simulink model "serial_leg"  (R2025b)
settings: Solver=ode15s  StartTime=0.0  StopTime=50  MaxStep=1e-3  RelTol=1e-3
undefined symbols (not defined in the file): X, Y, Z
libraries: sm_lib x106, nesl_utility x25, slpidlib x2
(part 1 of 3)
settings Model: Creator=Hhop  LastModifiedBy=13302
settings SolverCC: AlgebraicLoopSolver=TrustRegion  MinimalZcImpactIntegration=on
settings DebuggingCC: ReadBeforeWriteMsg=DisableAll  WriteAfterWriteMsg=DisableAll  WriteAfterReadMsg=DisableAll  MultiTaskDSMMsg=none
settings ModelReferenceCC: UpdateModelReferenceTargets=IfOutOfDate
settings SFSimCC: SFSimEcho=off
settings RTWCC: GPUComputeCapability=3.5  DLArmComputeVersion=19.05

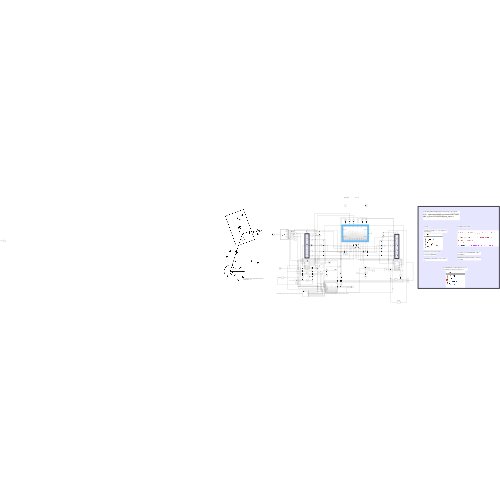
[thumbnail: Simulink's stored preview of the top-level diagram]
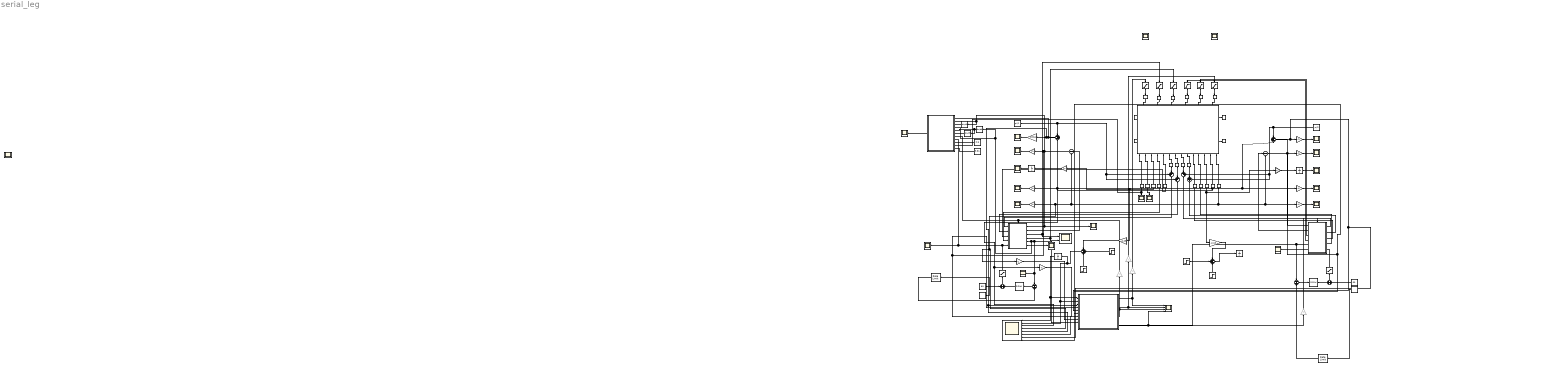
== system serial_leg ==
  note: 参考开源文档作者：韭菜的菜 链接：https://zhuanlan.zhihu.com/p/613007726 来源：知乎
  note: 图片来源 韭菜的菜 链接：https://zhuanlan.zhihu.com/p/613007726来源：知乎
  note: 运行步骤 :
  note: 所有开源文件必须置于同一文件夹(最好不要使用中文路径)
  note: 得到K参数后进入simulink 点击“运行”开始仿真
  note: addpath'(你所要想添加到的路径)'，具体用法可自行搜索
  note: 如果遇到如下图所示错误
  note: 可点击将其文件夹添加到MATLAB，或输入代码更换路径
  note: K = get_k_length(0.08)
  note: 在命令行窗口运行下图所示代码
  note: 如果想获取K矩阵关于腿长的函数的三次多项式系数在命令行窗口运行下图所示文件
  note: 该仿真是在b站轮腿机器人仿真开源上进行修改，链接：https://www.bilibili.com/read/cv26677904/?spm_id_from=333.999.0.0&jump_opus=1
  note: REAL serial/parallelogram mechanism: only A motors drive AD and AH. AD/AH use old upper-leg equivalent mass/inertia; DC/GHJ use old lower-leg equivalent mass/inertia. CEF and FG are transmission members with negligible mass. Original VMC and LQR are unchanged.
  Constant : Constant  Value=0.300
  Constant1 : Constant  Value=0.300
  Constant10 : Constant  Value=pi/2
  Constant12 : Constant  Value=pi/2
  Constant2 : Constant  Value=0.6
  Constant3 : Constant  Value=9.81
  Derivative : Derivative
  Derivative1 : Derivative
  Derivative2 : Derivative
  Gain : Gain  Gain=-0.08
  Gain1 : Gain  Gain=-0.05
  Gain{2..5} (4 alike) : Gain  Commented=through  Gain=-1
  Gain{22,24..26,33,36,38,40} (8 alike) : Gain  Gain=180/pi
  Gain29 : Gain  Gain=-0.0603
  Gain41 : Gain  Gain=-0.0603
  Gain6 : Gain  Gain=-1
  Gain7 : Gain  Gain=-1
  Integrator{1..4} (4 alike) : Integrator
  L_X : Scope
      settings: ActiveDisplayYMinimum=-0.7616  ActiveDisplayYMaximum=6.68295  DataLoggingVariableName=ScopeData7
  L_d_phi : Scope
      settings: ActiveDisplayYMinimum=-7.35816  ActiveDisplayYMaximum=0.81757  DataLoggingVariableName=ScopeData9
  L_d_theta : Scope
      settings: ActiveDisplayYMinimum=-21.72062  ActiveDisplayYMaximum=26.74747  DataLoggingVariableName=ScopeData13
  L_phi : Scope
      settings: ActiveDisplayYMinimum=-5.3646042462321226  ActiveDisplayYMaximum=10.928227501224146  DataLoggingVariableName=ScopeData22
  L_theta : Scope
      settings: ActiveDisplayYMinimum=-1.1015623623288358  ActiveDisplayYMaximum=1.79588161375989  DataLoggingVariableName=ScopeData25
  MATLAB Function : MATLAB Function  TreatAsAtomicUnit=on
  PID Controller2 : slpidlib/PID Controller  Controller=PID  Form=Parallel  TimeDomain=Continuous-time  UseExternalTs=off  SampleTime=-1  IntegratorMethod=Forward Euler  FilterMethod=Forward Euler  ControllerParametersSource=internal  P=500  I=0  UseKiTs=off  D=200  UseExternalDerivativeSource=off  N=100  UseFilter=on  TunerSelectOption=Transfer Function Based (PID Tuner App)  InitialConditionSource=internal  InitialConditionForIntegrator=0  InitialConditionForFilter=0  DifferentiatorICPrevScaledInput=0  ExternalReset=none  TrackingMode=off  Kt=1  LimitOutput=off  SatLimitsSource=internal  UpperSaturationLimit=inf  LowerSaturationLimit=-inf  LinearizeAsGain=on  AntiWindupMode=none  Kb=1  LimitIntegrator=off  UpperIntegratorSaturationLimit=inf  LowerIntegratorSaturationLimit=-inf  POutMin=[]  POutMax=[]  IOutMin=[]  IOutMax=[]  DOutMin=[]  DOutMax=[]  NOutMin=[]  NOutMax=[]  SumOutMin=[]  SumOutMax=[]  SaturationOutMin=[]  SaturationOutMax=[]  PParamMin=[]  PParamMax=[]  IParamMin=[]  IParamMax=[]  DParamMin=[]  DParamMax=[]  NParamMin=[]  NParamMax=[]  KbParamMin=[]  KbParamMax=[]  KtParamMin=[]  KtParamMax=[]  KbOutMin=[]  KbOutMax=[]  KtOutMin=[]  KtOutMax=[]  IntegratorOutMin=[]  IntegratorOutMax=[]  FilterOutMin=[]  FilterOutMax=[]  SumI1OutMin=[]  SumI1OutMax=[]  SumI2OutMin=[]  SumI2OutMax=[]  SumI3OutMin=[]  SumI3OutMax=[]  SumI4OutMin=[]  SumI4OutMax=[]  SumDOutMin=[]  SumDOutMax=[]  DifferentiatorOutMin=[]  DifferentiatorOutMax=[]  FilterDiffOutCoefMin=[]  FilterDiffOutCoefMax=[]  ReciprocalOutMin=[]  ReciprocalOutMax=[]  SumDenOutMin=[]  SumDenOutMax=[]  SumNumOutMin=[]  SumNumOutMax=[]  DivideOutMin=[]  DivideOutMax=[]  UdiffTsProdOutMin=[]  UdiffTsProdOutMax=[]  NTsProdOutMin=[]  NTsProdOutMax=[]  UintegralTsProdOutMin=[]  UintegralTsProdOutMax=[]  UngainTsProdOutMin=[]  UngainTsProdOutMax=[]  ClampingZeroOutDataTypeStr=Inherit: Inherit via back propagation  ClampingZeroOutMin=[]  ClampingZeroOutMax=[]  FilterDenConstantOutDataTypeStr=Inherit: Inherit via back propagation  FilterDenConstantOutMin=[]  FilterDenConstantOutMax=[]  PCopyOutDataTypeStr=Inherit: Inherit via back propagation  PCopyOutMin=[]  PCopyOutMax=[]  NCopyOutDataTypeStr=Inherit: Inherit via back propagation  NCopyOutMin=[]  NCopyOutMax=[]  IntegratorContinuousStateAttributes=''  IntegratorStateMustResolveToSignalObject=off  IntegratorRTWStateStorageClass=Auto  FilterContinuousStateAttributes=''  FilterStateMustResolveToSignalObject=off  FilterRTWStateStorageClass=Auto  ParallelPVariant=InternalParameters  IdealPVariant=Disabled  IVariant=InternalParameters  DVariant=InternalParameters  IntegratorVariant=Continuous  SatVariant=Disabled  AWVariant=Passthrough  PCopyVariant=Disabled  TRVariant=Disabled  FdbkBlocksVariant=Forward  IdealPFdbkVariant=Disabled  SatFdbkVariant=Disabled  DerivativeFilterVariant=ContFilter  NVariant=InternalParameters  NCopyVariant=Disabled  FilterICVariant=InternalICsFilter  IntegratorICVariant=InternalICs  ExternalResetVariant=Disabled  TRSumVariant=Passthrough  SumFdbkVariant=Disabled  SumVariant=Sum_PID  TsampFilterVariant=InternalTs  TsampNgainVariant=Passthrough  TsampIntegralVariant=Disabled_SignalSpec  ExternalSaturationOutDataTypeStr=Inherit: Same as second input  DerivativeSourceVariant=ErrorSignal  PreIntVariant=InternalPreInt
  PID Controller3 : slpidlib/PID Controller  Controller=PID  Form=Parallel  TimeDomain=Continuous-time  UseExternalTs=off  SampleTime=-1  IntegratorMethod=Forward Euler  FilterMethod=Forward Euler  ControllerParametersSource=internal  P=500  I=0  UseKiTs=off  D=200  UseExternalDerivativeSource=off  N=100  UseFilter=on  TunerSelectOption=Transfer Function Based (PID Tuner App)  InitialConditionSource=internal  InitialConditionForIntegrator=0  InitialConditionForFilter=0  DifferentiatorICPrevScaledInput=0  ExternalReset=none  TrackingMode=off  Kt=1  LimitOutput=off  SatLimitsSource=internal  UpperSaturationLimit=inf  LowerSaturationLimit=-inf  LinearizeAsGain=on  AntiWindupMode=none  Kb=1  LimitIntegrator=off  UpperIntegratorSaturationLimit=inf  LowerIntegratorSaturationLimit=-inf  POutMin=[]  POutMax=[]  IOutMin=[]  IOutMax=[]  DOutMin=[]  DOutMax=[]  NOutMin=[]  NOutMax=[]  SumOutMin=[]  SumOutMax=[]  SaturationOutMin=[]  SaturationOutMax=[]  PParamMin=[]  PParamMax=[]  IParamMin=[]  IParamMax=[]  DParamMin=[]  DParamMax=[]  NParamMin=[]  NParamMax=[]  KbParamMin=[]  KbParamMax=[]  KtParamMin=[]  KtParamMax=[]  KbOutMin=[]  KbOutMax=[]  KtOutMin=[]  KtOutMax=[]  IntegratorOutMin=[]  IntegratorOutMax=[]  FilterOutMin=[]  FilterOutMax=[]  SumI1OutMin=[]  SumI1OutMax=[]  SumI2OutMin=[]  SumI2OutMax=[]  SumI3OutMin=[]  SumI3OutMax=[]  SumI4OutMin=[]  SumI4OutMax=[]  SumDOutMin=[]  SumDOutMax=[]  DifferentiatorOutMin=[]  DifferentiatorOutMax=[]  FilterDiffOutCoefMin=[]  FilterDiffOutCoefMax=[]  ReciprocalOutMin=[]  ReciprocalOutMax=[]  SumDenOutMin=[]  SumDenOutMax=[]  SumNumOutMin=[]  SumNumOutMax=[]  DivideOutMin=[]  DivideOutMax=[]  UdiffTsProdOutMin=[]  UdiffTsProdOutMax=[]  NTsProdOutMin=[]  NTsProdOutMax=[]  UintegralTsProdOutMin=[]  UintegralTsProdOutMax=[]  UngainTsProdOutMin=[]  UngainTsProdOutMax=[]  ClampingZeroOutDataTypeStr=Inherit: Inherit via back propagation  ClampingZeroOutMin=[]  ClampingZeroOutMax=[]  FilterDenConstantOutDataTypeStr=Inherit: Inherit via back propagation  FilterDenConstantOutMin=[]  FilterDenConstantOutMax=[]  PCopyOutDataTypeStr=Inherit: Inherit via back propagation  PCopyOutMin=[]  PCopyOutMax=[]  NCopyOutDataTypeStr=Inherit: Inherit via back propagation  NCopyOutMin=[]  NCopyOutMax=[]  IntegratorContinuousStateAttributes=''  IntegratorStateMustResolveToSignalObject=off  IntegratorRTWStateStorageClass=Auto  FilterContinuousStateAttributes=''  FilterStateMustResolveToSignalObject=off  FilterRTWStateStorageClass=Auto  ParallelPVariant=InternalParameters  IdealPVariant=Disabled  IVariant=InternalParameters  DVariant=InternalParameters  IntegratorVariant=Continuous  SatVariant=Disabled  AWVariant=Passthrough  PCopyVariant=Disabled  TRVariant=Disabled  FdbkBlocksVariant=Forward  IdealPFdbkVariant=Disabled  SatFdbkVariant=Disabled  DerivativeFilterVariant=ContFilter  NVariant=InternalParameters  NCopyVariant=Disabled  FilterICVariant=InternalICsFilter  IntegratorICVariant=InternalICs  ExternalResetVariant=Disabled  TRSumVariant=Passthrough  SumFdbkVariant=Disabled  SumVariant=Sum_PID  TsampFilterVariant=InternalTs  TsampNgainVariant=Passthrough  TsampIntegralVariant=Disabled_SignalSpec  ExternalSaturationOutDataTypeStr=Inherit: Same as second input  DerivativeSourceVariant=ErrorSignal  PreIntVariant=InternalPreInt
  PS-Simulink Converter{1,18..22,24,27..37} (18 alike) : nesl_utility/PS-Simulink Converter  PhysicalDomain=network_engine_domain  SubClassName=ps_output  LeftPortType=input  RightPortType=output  PseudoPeriodic=off  Frequencies=[]  VectorFormat=1-D array  Unit=inherit  AffineConversion=off
  R_X : Scope
      settings: ActiveDisplayYMinimum=-0.79846  ActiveDisplayYMaximum=7.01473  DataLoggingVariableName=ScopeData8
  R_d_phi : Scope
      settings: ActiveDisplayYMinimum=-7.35816  ActiveDisplayYMaximum=0.81757  DataLoggingVariableName=ScopeData11
  R_d_theta : Scope
      settings: ActiveDisplayYMinimum=-51.86845  ActiveDisplayYMaximum=175.83384  DataLoggingVariableName=ScopeData14
  R_phi : Scope
      settings: ActiveDisplayYMinimum=-1.27659  ActiveDisplayYMaximum=11.48927  DataLoggingVariableName=ScopeData17
  R_theta : Scope
      settings: ActiveDisplayYMinimum=-20.84145  ActiveDisplayYMaximum=19.50938  DataLoggingVariableName=ScopeData26
  RampH : RateLimiter  RisingSlewLimit=0.15  FallingSlewLimit=-0.15  SampleTimeMode=inherited  InitialCondition=0.15
  RampH1 : RateLimiter  RisingSlewLimit=0.15  FallingSlewLimit=-0.15  SampleTimeMode=inherited  InitialCondition=0.15
  Saturation{1..4} (4 alike) : Saturate  UpperLimit=15  LowerLimit=-15
  Saturation5 : Saturate  UpperLimit=300  LowerLimit=-300
  Saturation6 : Saturate  UpperLimit=300  LowerLimit=-300
  Saturation7 : Saturate  UpperLimit=6.5  LowerLimit=-6.5
  Saturation8 : Saturate  UpperLimit=6.5  LowerLimit=-6.5
  Scope : Scope  NumInputPorts=4
      settings: ActiveDisplayYMinimum=-12.472520998947731  ActiveDisplayYMaximum=6.2920167785247285
  Scope{1,3,5..12} (10 alike) : Scope
      Scope1 settings: ActiveDisplayYMinimum=-9.10613  ActiveDisplayYMaximum=7.92497
      Scope10 settings: ActiveDisplayYMinimum=-1  ActiveDisplayYMaximum=1  DataLoggingVariableName=ScopeData18
      Scope11 settings: ActiveDisplayYMinimum=-76.924531638657356  ActiveDisplayYMaximum=319.01997172873973  DataLoggingVariableName=ScopeData19
      Scope12 settings: ActiveDisplayYMinimum=-61.263322403911886  ActiveDisplayYMaximum=340.14036915599019  DataLoggingVariableName=ScopeData20
      Scope3 settings: ActiveDisplayYMinimum=0.1339320623544637  ActiveDisplayYMaximum=0.31073823748944696  DataLoggingVariableName=ScopeData3
      Scope5 settings: ActiveDisplayYMinimum=1.4730644438405058  ActiveDisplayYMaximum=1.6436882527053356  DataLoggingVariableName=ScopeData5
      Scope6 settings: ActiveDisplayYMinimum=-2.43035  ActiveDisplayYMaximum=2.35376  DataLoggingVariableName=ScopeData6
      Scope7 settings: DataLoggingVariableName=ScopeData10
      Scope8 settings: DataLoggingVariableName=ScopeData12
      Scope9 settings: ActiveDisplayYMinimum=-45.163347629745211  ActiveDisplayYMaximum=67.7915265425867  DataLoggingVariableName=ScopeData15
  Scope2 : Scope  NumInputPorts=8
      settings: ActiveDisplayYMinimum=-0.30331626838987974  ActiveDisplayYMaximum=0.2904853430526374  DataLoggingVariableName=ScopeData2
  Scope4 : Scope  NumInputPorts=2
      settings: ActiveDisplayYMinimum=-44.227576016086928  ActiveDisplayYMaximum=17.910617583564356  DataLoggingVariableName=ScopeData4
  Simulink-PS Converter{1..6} (6 alike) : nesl_utility/Simulink-PS Converter  PhysicalDomain=network_engine_domain  SubClassName=ps_input  LeftPortType=input  RightPortType=output  PseudoPeriodic=off  Frequencies=[]  NoiseDistribution=none  NoiseParameters=[]  Unit=1  AffineConversion=off  FilteringAndDerivatives=provide  SimscapeFilterOrder=1  InputFilterTimeConstant=0.001  UdotUserProvided=0
  Step1 : Step  Time=2  After=0.5  SampleTime=0
  Step5 : Step  Time=5  After=0.5  SampleTime=0
  Step6 : Step  Time=5  After=0.5  SampleTime=0
  Step7 : Step  Time=2  After=0.5  SampleTime=0
  Subsystem : Subsystem
  Subsystem4 : Subsystem
      settings: PortSchema="{\"entries\":[{\"content\":{\"sides\":[{\"content\":{\"connectorIds\":[\"In1\",\"In2\",\"In3\",\"In4\",\"In5\"]},\"type\":\"ConnectorPlacement.EquallySpacedRectSide\",\"uuid\":\"40de31e0-cc19-460f-99e9-affbb47f7204\"},{\"content\":{\"connectorIds\":[\"Out1\",\"Out2\",\"Out3\",\"Out4\",\"Out5\",\"Out6\"],\"side\":\"RIGHT\"},\"type\":\"ConnectorPlacement.EquallySpacedRectSide\",\"uuid\":\"e61df4ab-633d-456a-aa2d-223df880274d\"},{\"content\":{\"connectorIds\":[\"In6\"],\"side\":\"TOP\"},\"type\":\"ConnectorPlacement.EquallySpacedRectSide\",\"uuid\":\"a7334146-3144-4ab1-9f08-8bf1583597b4\"}]},\"type\":\"ConnectorPlacement.EquallySpacedConnector\",\"uuid\":\"1490fe93-b025-4c86-96e6-b1bfc13c7f50\"}],\"packageUris\":[\"http://schema.mathworks.com/mf0/Connector/R2020b\"],\"version\":\"1.0\"}"
  Sum1 : Sum  Inputs=+-+
  Sum13 : Sum  Inputs=++|
  Sum14 : Sum  Inputs=|++
  Sum15 : Sum  Inputs=|++
  Sum16 : Sum  Inputs=|--
  Sum17 : Sum  Inputs=+--
  Sum18 : Sum  Inputs=+|+
  Sum2 : Sum  Inputs=+-+
  Sum20 : Sum  Inputs=++|
  Sum23 : Sum  Inputs=-|+
  Sum24 : Sum  Inputs=+--
  Sum25 : Sum  Inputs=+|+
  Sum27 : Sum  Inputs=|--
  Sum29 : Sum  Inputs=-|+
  blance_leg_model : Subsystem
      settings: PortSchema="{\"entries\":[{\"content\":{\"sides\":[{\"content\":{\"connectorIds\":[\"LConn1\",\"LConn2\",\"LConn3\",\"LConn4\",\"LConn5\",\"LConn6\"]},\"type\":\"ConnectorPlacement.EquallySpacedRectSide\",\"uuid\":\"df2d0b15-ec70-4430-8d90-67c6d88950b4\"},{\"content\":{\"connectorIds\":[\"RConn1\",\"RConn2\",\"RConn3\",\"RConn4\",\"RConn5\",\"RConn6\",\"RConn7\",\"RConn8\",\"RConn9\",\"RConn10\",\"RConn11\",\"RConn12\",\"RConn13\",\"RConn14\"],\"side\":\"RIGHT\"},\"type\":\"ConnectorPlacement.EquallySpacedRectSide\",\"uuid\":\"ec9b4787-d265-4ad9-b676-e253d2304993\"},{\"content\":{\"connectorIds\":[\"LConn7\",\"LConn8\"],\"side\":\"TOP\"},\"type\":\"ConnectorPlacement.EquallySpacedRectSide\",\"uuid\":\"40dd08fe-dc32-4cee-bbb8-c1ec6d04ee32\"},{\"content\":{\"connectorIds\":[\"RConn15\",\"RConn16\"],\"side\":\"BOTTOM\"},\"type\":\"ConnectorPlacement.EquallySpacedRectSide\",\"uuid\":\"0f9c1faf-3e52-4dca-bbb1-0993be9fa88c\"}]},\"type\":\"ConnectorPlacement.EquallySpacedConnector\",\"uuid\":\"d540d646-85aa-4f97-ae4d-1bccec971368\"}],\"packageUris\":[\"http://schema.mathworks.com/mf0/Connector/R2020b\"],\"version\":\"1.0\"}"
  control : Subsystem
      settings: PortSchema="{\"entries\":[{\"content\":{\"sides\":[{\"content\":{\"connectorIds\":[\"In1\",\"In2\",\"In3\",\"In4\",\"In5\"]},\"type\":\"ConnectorPlacement.EquallySpacedRectSide\",\"uuid\":\"40de31e0-cc19-460f-99e9-affbb47f7204\"},{\"content\":{\"connectorIds\":[\"Out1\",\"Out2\",\"Out3\",\"Out4\",\"Out5\",\"Out6\"],\"side\":\"RIGHT\"},\"type\":\"ConnectorPlacement.EquallySpacedRectSide\",\"uuid\":\"e61df4ab-633d-456a-aa2d-223df880274d\"},{\"content\":{\"connectorIds\":[\"In6\"],\"side\":\"TOP\"},\"type\":\"ConnectorPlacement.EquallySpacedRectSide\",\"uuid\":\"a7334146-3144-4ab1-9f08-8bf1583597b4\"}]},\"type\":\"ConnectorPlacement.EquallySpacedConnector\",\"uuid\":\"1490fe93-b025-4c86-96e6-b1bfc13c7f50\"}],\"packageUris\":[\"http://schema.mathworks.com/mf0/Connector/R2020b\"],\"version\":\"1.0\"}"
  mean_x2 : Scope
      settings: ActiveDisplayYMinimum=-0.05008  ActiveDisplayYMaximum=0.21605  DataLoggingVariableName=ScopeData16
  除去轮子后机体重量 : Constant  Value=60
  除去轮子后机体重量， : Constant  Value=60
  wires:
  Integrator4/1 -> R_X/1  "x"
  Integrator2/1 -> L_X/1  "x"
  除去轮子后机体重量，/1 -> Sum25/1
  Sum27/1 -> Scope2/8, Subsystem/6(dthetaR), Gain25/1
  Gain40/1 -> L_d_phi/1
  Gain24/1 -> R_theta/1
  Gain38/1 -> L_d_theta/1
  Constant12/1 -> Sum15/2, Sum14/2, Sum17/1
  Sum29/1 -> PID Controller3/1
  Gain33/1 -> R_phi/1
  Gain36/1 -> L_theta/1
  Gain41/1 -> Integrator2/1  "x'"
  Sum16/1 -> Derivative/1, MATLAB Function/2(theta_dot), Subsystem/4(dthetaL), Scope2/6, Gain38/1
  Gain26/1 -> R_d_phi/1
  Gain22/1 -> L_phi/1
  Constant10/1 -> Sum20/1, Sum13/1, Sum24/1
  Gain29/1 -> Integrator4/1  "x'"
  Sum23/1 -> PID Controller2/1
  PID Controller2/1 -> Sum25/2
  Sum17/1 -> Subsystem/5(thetaR), Scope2/7, Gain24/1
  Gain25/1 -> R_d_theta/1
  除去轮子后机体重量/1 -> Sum18/2
  PID Controller3/1 -> Sum18/1
  PS-Simulink Converter32/1 -> Sum13/2
  PS-Simulink Converter35/1 -> Sum15/1
  PS-Simulink Converter33/1 -> Sum14/1
  PS-Simulink Converter34/1 -> Sum20/2
  Sum13/1 -> control/1(phi1)
  Sum20/1 -> control/2(phi4)
  Sum14/1 -> Subsystem4/1(phi1)
  Sum15/1 -> Subsystem4/2(phi4)
  PS-Simulink Converter31/1 -> control/3(d_phi1)
  PS-Simulink Converter29/1 -> control/4(d_phi4)
  PS-Simulink Converter20/1 -> Subsystem4/3(d_phi1)
  PS-Simulink Converter21/1 -> Subsystem4/4(d_phi4)
  PS-Simulink Converter28/1 -> Gain41/1, Gain1/1
  PS-Simulink Converter22/1 -> Gain29/1, Gain/1
  PS-Simulink Converter1/1 -> Gain33/1, Sum17/3, Gain7/1, Scope2/3, Gain22/1, Sum24/3
  PS-Simulink Converter24/1 -> Gain6/1, Scope2/4, Gain40/1, Sum16/2, Gain26/1, Sum27/2
  control/5(L0) -> Subsystem/9(L_left), Scope3/1, Sum23/1, Derivative1/1, MATLAB Function/4(L0)
  control/1(phi0) -> Scope5/1, Sum24/2
  control/2(d_phi0) -> Sum16/1
  Subsystem4/2(d_phi0) -> Sum27/1
  Subsystem4/5(L0) -> Sum29/1, Subsystem/10(L_right)
  Sum18/1 -> Saturation5/1
  Sum25/1 -> Saturation6/1
  Saturation6/1 -> MATLAB Function/8(F), Scope12/1, control/5(F0)
  control/3(T1) -> Scope4/1, Saturation1/1
  Subsystem4/3(T1) -> Saturation4/1
  control/4(T2) -> Scope4/2, Saturation2/1
  Subsystem4/4(T2) -> Saturation3/1
  Integrator3/1 -> Subsystem/1(X), Scope2/1
  Gain1/1 -> Sum1/1
  Sum1/1 -> Scope2/2, Subsystem/2(dX), Integrator3/1
  Gain/1 -> Sum2/1
  Sum2/1 -> Integrator1/1
  Step1/1 -> Sum1/2
  Step5/1 -> Sum1/3
  Step7/1 -> Sum2/2
  Step6/1 -> Sum2/3
  Saturation5/1 -> Subsystem4/5(F0)
  Sum24/1 -> MATLAB Function/1(theta), Subsystem/3(thetaL), Scope2/5, Gain36/1
  Subsystem/1(Tw_L) -> Gain2/1, Scope/1
  Subsystem/2(Tw_R) -> Scope/2, Gain3/1
  Subsystem/3(Tp_L) -> Scope/3, Gain4/1
  Subsystem/4(Tp_R) -> Scope/4, Gain5/1
  Gain2/1 -> Saturation7/1
  Gain3/1 -> Saturation8/1
  Gain4/1 -> MATLAB Function/7(Tp), control/6(Tp)
  Gain5/1 -> Subsystem4/6(Tp)
  Gain6/1 -> Subsystem/8(dtheta)
  Gain7/1 -> Subsystem/7(theta)
  control/6(phi) -> Scope7/1
  Subsystem4/6(phi) -> Scope8/1
  Derivative/1 -> MATLAB Function/3(theta_ddot)
  Derivative1/1 -> Derivative2/1, MATLAB Function/5(L0_dot)
  Derivative2/1 -> MATLAB Function/6(L0_ddot)
  Constant2/1 -> MATLAB Function/9(m_omega)
  Constant3/1 -> MATLAB Function/11(g)
  PS-Simulink Converter18/1 -> MATLAB Function/10(zM_ddot), Scope9/1
  PS-Simulink Converter19/1 -> Scope10/1
  MATLAB Function/1(Fn) -> Scope11/1
  Constant/1 -> RampH/1
  RampH/1 -> Sum29/2
  Constant1/1 -> RampH1/1
  RampH1/1 -> Sum23/2
  Subsystem4/1(phi0) -> Sum17/2
  Saturation1/1 -> Simulink-PS Converter1/1
  Saturation2/1 -> Simulink-PS Converter3/1
  Saturation3/1 -> Simulink-PS Converter2/1
  Saturation4/1 -> Simulink-PS Converter5/1
  Saturation7/1 -> Simulink-PS Converter6/1
  Saturation8/1 -> Simulink-PS Converter4/1
  connections:
  blance_leg_model/LConn2 -- Simulink-PS Converter1/RConn1
  blance_leg_model/LConn3 -- Simulink-PS Converter3/RConn1
  blance_leg_model/LConn4 -- Simulink-PS Converter2/RConn1
  blance_leg_model/LConn5 -- Simulink-PS Converter5/RConn1
  blance_leg_model/RConn10 -- PS-Simulink Converter20/LConn1
  blance_leg_model/RConn11 -- PS-Simulink Converter21/LConn1
  blance_leg_model/RConn2 -- PS-Simulink Converter19/LConn1
  blance_leg_model/RConn12 -- PS-Simulink Converter22/LConn1
  blance_leg_model/RConn3 -- PS-Simulink Converter28/LConn1
  blance_leg_model/RConn14 -- PS-Simulink Converter24/LConn1
  blance_leg_model/RConn5 -- PS-Simulink Converter31/LConn1
  blance_leg_model/RConn1 -- PS-Simulink Converter18/LConn1
  blance_leg_model/RConn4 -- PS-Simulink Converter29/LConn1
  blance_leg_model/RConn13 -- PS-Simulink Converter1/LConn1
  blance_leg_model/RConn6 -- PS-Simulink Converter32/LConn1
  blance_leg_model/RConn7 -- PS-Simulink Converter34/LConn1
  blance_leg_model/RConn8 -- PS-Simulink Converter33/LConn1
  blance_leg_model/RConn9 -- PS-Simulink Converter35/LConn1
  blance_leg_model/LConn7 -- PS-Simulink Converter27/LConn1
  blance_leg_model/LConn8 -- PS-Simulink Converter30/LConn1
  blance_leg_model/RConn15 -- PS-Simulink Converter36/LConn1
  blance_leg_model/RConn16 -- PS-Simulink Converter37/LConn1
  blance_leg_model/LConn1 -- Simulink-PS Converter6/RConn1
  blance_leg_model/LConn6 -- Simulink-PS Converter4/RConn1

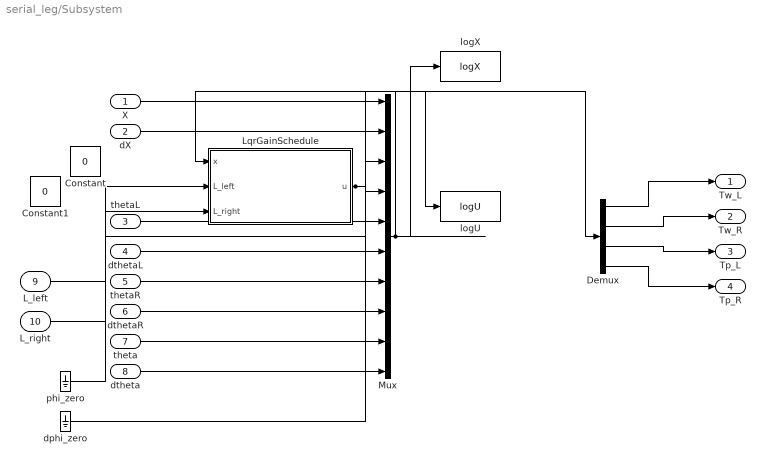
== system serial_leg/Subsystem ==
  X : Inport
  dX : Inport  Port=2
  thetaL : Inport  Port=3
  dthetaL : Inport  Port=4
  thetaR : Inport  Port=5
  dthetaR : Inport  Port=6
  theta : Inport  Port=7
  dtheta : Inport  Port=8
  L_left : Inport  Port=9
  L_right : Inport  Port=10
  Constant : Constant  Value=0
  Constant1 : Constant  Value=0
  Demux : Demux
  LqrGainSchedule : MATLAB Function  TreatAsAtomicUnit=on
  Mux : Mux  Inputs=10
  dphi_zero : Ground
  logU : ToWorkspace  VariableName=logU  SaveFormat=Structure With Time  SampleTime=-1
  logX : ToWorkspace  VariableName=logX  SaveFormat=Structure With Time  SampleTime=-1
  phi_zero : Ground
  Tw_L : Outport
  Tw_R : Outport  Port=2
  Tp_L : Outport  Port=3
  Tp_R : Outport  Port=4
  wires:
  Mux/1 -> LqrGainSchedule/1(x), logX/1
  Demux/1 -> Tw_L/1
  Demux/2 -> Tw_R/1
  Demux/3 -> Tp_L/1
  Demux/4 -> Tp_R/1
  X/1 -> Mux/1
  dX/1 -> Mux/2
  thetaL/1 -> Mux/5
  dthetaL/1 -> Mux/6
  thetaR/1 -> Mux/7
  dthetaR/1 -> Mux/8
  theta/1 -> Mux/9
  dtheta/1 -> Mux/10
  L_left/1 -> LqrGainSchedule/2(L_left)
  L_right/1 -> LqrGainSchedule/3(L_right)
  LqrGainSchedule/1(u) -> Demux/1, logU/1
  phi_zero/1 -> Mux/3
  dphi_zero/1 -> Mux/4

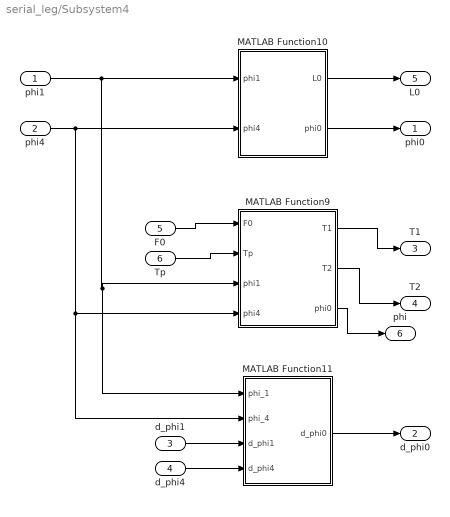
== system serial_leg/Subsystem4 ==
  phi1 : Inport
  phi4 : Inport  Port=2
  d_phi1 : Inport  Port=3
  d_phi4 : Inport  Port=4
  F0 : Inport  Port=5
  Tp : Inport  Port=6
  MATLAB Function10 : MATLAB Function  TreatAsAtomicUnit=on
  MATLAB Function11 : MATLAB Function  TreatAsAtomicUnit=on
  MATLAB Function9 : MATLAB Function  TreatAsAtomicUnit=on
  phi0 : Outport
  d_phi0 : Outport  Port=2
  T1 : Outport  Port=3
  T2 : Outport  Port=4
  L0 : Outport  Port=5
  phi : Outport  Port=6
  wires:
  phi1/1 -> MATLAB Function11/1(phi_1), MATLAB Function9/3(phi1), MATLAB Function10/1(phi1)
  MATLAB Function10/2(phi0) -> phi0/1
  MATLAB Function11/1(d_phi0) -> d_phi0/1
  Tp/1 -> MATLAB Function9/2(Tp)
  d_phi4/1 -> MATLAB Function11/4(d_phi4)
  d_phi1/1 -> MATLAB Function11/3(d_phi1)
  MATLAB Function9/1(T1) -> T1/1
  phi4/1 -> MATLAB Function11/2(phi_4), MATLAB Function9/4(phi4), MATLAB Function10/2(phi4)
  F0/1 -> MATLAB Function9/1(F0)
  MATLAB Function9/2(T2) -> T2/1
  MATLAB Function10/1(L0) -> L0/1
  MATLAB Function9/3(phi0) -> phi/1
